simulink model "vita_sys_03"  (R2025b)
settings: Solver=VariableStepAuto  StartTime=0.0  StopTime=15.0  RelTol=1e-3
undefined symbols (not defined in the file): matlabshared
libraries: drivingscenarioandsensors x2, drivinglib x1
settings Model: Creator=ADMIIN  LastModifiedBy=ADMIIN

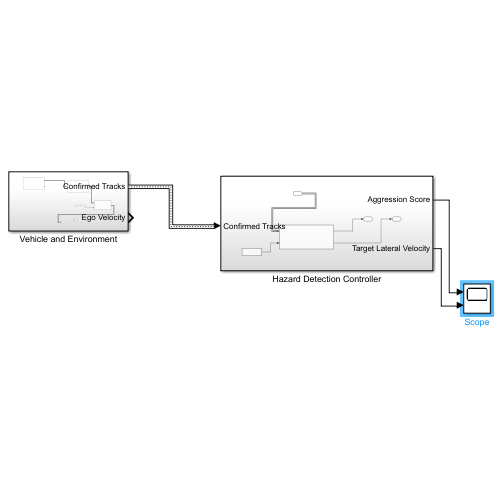
[thumbnail: Simulink's stored preview of the top-level diagram]
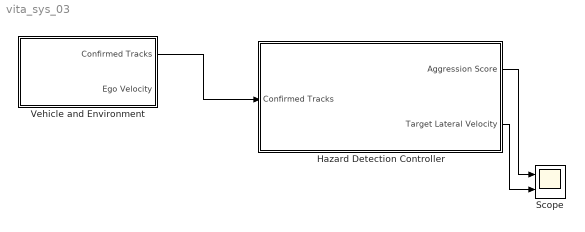
== system vita_sys_03 ==
  Hazard Detection Controller : Subsystem
  Scope : Scope  NumInputPorts=2
      settings: ActiveDisplayYMinimum=-7.5657065421200151  ActiveDisplayYMaximum=9.1854960154626184
  Vehicle and Environment : Subsystem
  wires:
  Vehicle and Environment/1(Confirmed Tracks) -> Hazard Detection Controller/1(Confirmed Tracks)
  Hazard Detection Controller/1(Aggression Score) -> Scope/1
  Hazard Detection Controller/2(Target Lateral Velocity) -> Scope/2

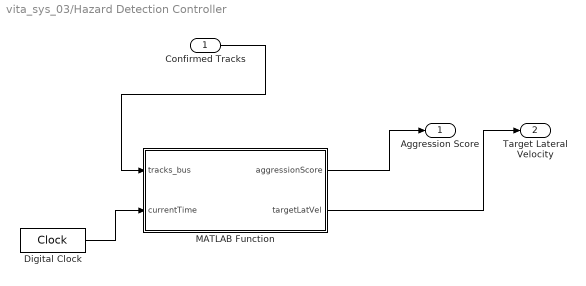
== system vita_sys_03/Hazard Detection Controller ==
  Confirmed Tracks : Inport
  Digital Clock : DigitalClock
  MATLAB Function : MATLAB Function  TreatAsAtomicUnit=on
  Aggression Score : Outport
  Target Lateral Velocity : Outport  Port=2
  wires:
  Confirmed Tracks/1 -> MATLAB Function/1(tracks_bus)
  MATLAB Function/1(aggressionScore) -> Aggression Score/1
  MATLAB Function/2(targetLatVel) -> Target Lateral Velocity/1
  Digital Clock/1 -> MATLAB Function/2(currentTime)

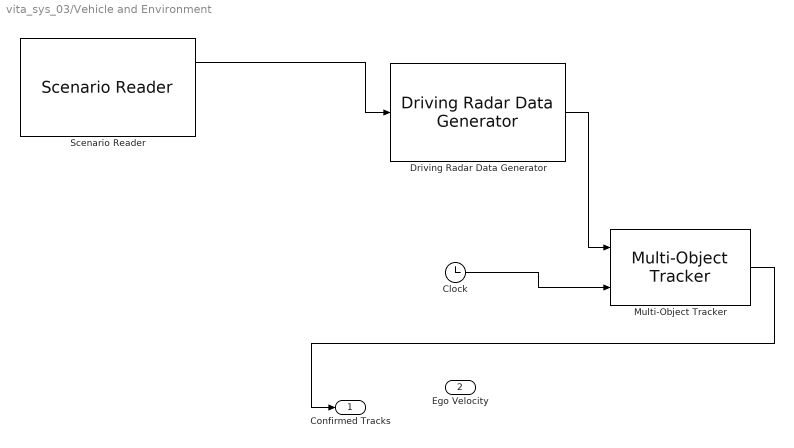
== system vita_sys_03/Vehicle and Environment ==
  Clock : Clock
  Driving Radar Data Generator : drivingscenarioandsensors/Driving Radar Data Generator  SensorIndex=1  UpdateRate=10  MountingLocation=[ 3.4, 0, 0.2 ]  MountingAngles=[0 0 0]  HasElevation=on  HasRangeRate=off  HasNoise=on  HasFalseAlarms=on  HasOcclusion=on  MaxNumReportsSource=Property  MaxNumReports=50  TargetReportFormat=Clustered detections  DetectionCoordinates=Body  TrackCoordinates=Body  BusNameSource=Auto  BusName=BusDrivingRadarDataGenerator  SimulateUsing=Interpreted execution  AzimuthResolution=4  ElevationResolution=5  RangeResolution=2.5  RangeRateResolution=0.5  AzimuthBiasFraction=0.1  ElevationBiasFraction=0.1  RangeBiasFraction=0.05  RangeRateBiasFraction=0.05  FieldOfView=[ 20, 5 ]  RangeLimits=[ 0, 150 ]  RangeRateLimits=[ -100, 100 ]  DetectionProbability=0.9  FalseAlarmRate=1e-06  ReferenceRange=100  ReferenceRCS=0  CenterFrequency=77e9  FilterInitializationFcn=initcvekf  ConfirmationThreshold=[2 3]  DeletionThreshold=[5 5]  InitialSeedSource=Repeatable  InitialSeed=0  UsedSeed=matlabshared.tracking.internal.SimulinkUtilities.seedManager(gcb)  ProfilesSource=From Scenario Reader block  ProfilesParameters=driving.internal.ActorProfilesRadarParameters  ProfilesExpression=struct('ClassID',0,'Length',4.7,'Width',1.8,'Height',1.4,'OriginOffset',[-1.35 0 0],'RCSPattern',[10 10;10 10],'RCSAzimuthAngles',[-180 180],'RCSElevationAngles',[-90 90])
  Multi-Object Tracker : drivinglib/Multi-Object Tracker  TrackerIndex=uint32( 0 )  FilterInitializationFcn=initcvkf  AssignmentThreshold=30.0  ConfirmationThreshold=[ 2, 3 ]  DeletionThreshold=[ 5, 5 ]  MaxNumTracks=200  MaxNumSensors=20  OOSMHandling=Terminate  StateParametersSimulink=struct  HasStateParametersInput=off  TimeInputSource=Input port  HasCostMatrixInput=off  HasDetectableTrackIDsInput=off  BusNameSource=Auto  BusName=BusMultiObjectTracker  TentativeTracksOutputPort=off  AllTracksOutputPort=off  SimulateUsing=Interpreted execution
  Scenario Reader : drivingscenarioandsensors/Scenario Reader  ScenarioSource=From file  ScenarioFileName=E:\tata\aggression_scenario.mat  ScenarioVariableName=scenario  OutputCoordinateSystem=Vehicle coordinates  EgoVehicleSource=Scenario  EgoVehicleActorID=1  OrientVehiclesOnRoad=off  OutputEgoVehiclePose=on  OutputEgoVehicleState=off  SampleTime=0.1  LaneBoundaryOutput=None  LaneBoundaryDistance=0:0.5:9.5  LaneBoundaryLocation=Center of lane markings  BusNameSource=Auto  BusName=BusActors  BusNumActorsSource=Scenario  BusNumActors=100  BusName2Source=Auto  BusName2=BusLaneBoundaries  BusNumLaneBoundariesSource=Scenario  BusNumLaneBoundaries=10  BusName3Source=Auto  BusName3=BusEgoActor  BusName4Source=Auto  BusName4=BusEgoState  ShowCoordinateLabels=on  SimulateUsing=Interpreted execution
  Confirmed Tracks : Outport
  Ego Velocity : Outport  Port=2
  wires:
  Scenario Reader/1 -> Driving Radar Data Generator/1
  Multi-Object Tracker/1 -> Confirmed Tracks/1
  Driving Radar Data Generator/1 -> Multi-Object Tracker/1
  Clock/1 -> Multi-Object Tracker/2

== matlab function vita_sys_03/Hazard Detection Controller/MATLAB Function ==
  data: tracks_bus input; aggressionScore output; targetLatVel output; currentTime input
function [aggressionScore, targetLatVel] = fcn(tracks_bus, currentTime)
% This function analyzes vehicle tracks to detect aggressive driving.

% Persistent variables hold their value between simulation steps
persistent score prevTime;

% Initialize persistent variables on the first run
if isempty(score)
    score = 0;
    prevTime = 0;
end

% Default outputs
aggressionScore = score;
targetLatVel = 0;

% Find the closest track in front of the ego car
closestDist = 150; % Max distance to check
leadCarTrackExists = false;

% The input 'tracks_bus' contains NumTracks and an array Tracks
% We must loop from 1 to the number of valid tracks.
for i = 1:tracks_bus.NumTracks
    
    % Access the i-th track from the 'Tracks' array inside the bus
    currentTrack = tracks_bus.Tracks(i);
    
    % The state vector is in a field named 'State'
    % State has [x; vx; y; vy; ...]
    pos = currentTrack.State([1,3]); % [x,y] position
    dist = norm(pos);
    
    if pos(1) > 2 && dist < closestDist % Check if it's in front and closest
        closestDist = dist;
        vel = currentTrack.State([2,4]); % [vx, vy] velocity
        targetLatVel = vel(2);
        leadCarTrackExists = true;
    end
end

dt = currentTime - prevTime;

% Analyze the lead car's behavior if it exists and time has passed
if leadCarTrackExists && dt > 0.1
    
    % Check for high lateral velocity (swerving)
    if abs(targetLatVel) > 3.5 % Threshold for aggressive swerve (m/s)
        score = score + 5; % Add points for swerving
    end
    
    % Update state for next time step
    prevTime = currentTime;
end

aggressionScore = score;

end
